simulink model "pam_enlace_simulink"  (R2026a)
settings: Solver=ode23tb  StopTime=T_sim  MaxStep=1e-6  RelTol=1e-4
PostLoadFcn:
  | run(fullfile(fileparts(get_param(bdroot,'FileName')),'pam_simulink_init.m'))
InitFcn:
  | run(fullfile(fileparts(get_param(bdroot,'FileName')),'pam_simulink_init.m'))
values from neighbouring files (symbols this model uses):
  bc = cal.bc    [pam_simulink_init.m]
  den_canal = P.den    [pam_simulink_init.m]
  hc = fliplr(pc) / Ec    [pam_simulink_init.m]
  num_canal = P.num    [pam_simulink_init.m]
  t0 = 3.125e-6    (= 3.125e-06)    [pam_simulink_init.m]
  t_fim = t0 + 7*Tsa    [pam_simulink_init.m]
  t_kstar = t0 + kstar*Tsa    [pam_simulink_init.m]
  tab_bits = zeros(4)    [pam_simulink_init.m]
  thr_u = [cal.thr_u, inf(1, 3 - numel(cal.thr_u))]    [pam_simulink_init.m]
  thr_z = [cal.thr_z, inf(1, 3 - numel(cal.thr_z))]    [pam_simulink_init.m]
  Ts = P.Ts    [pam_simulink_init.m]
  Tsa = P.Tsa    [pam_simulink_init.m]
  Vmax = 3.3    [pam_simulink_init.m]
  Vref = 3.3    [pam_simulink_init.m]
undefined symbols (not defined in the file or in its folder): M, sigma_ruido
settings Model: Creator=fonfon  LastModifiedBy=fonfon

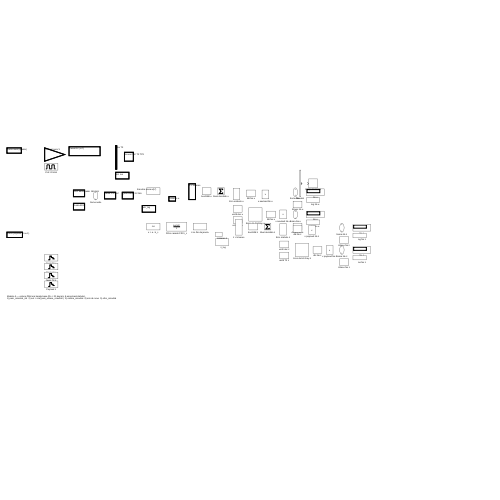
[thumbnail: Simulink's stored preview of the top-level diagram]
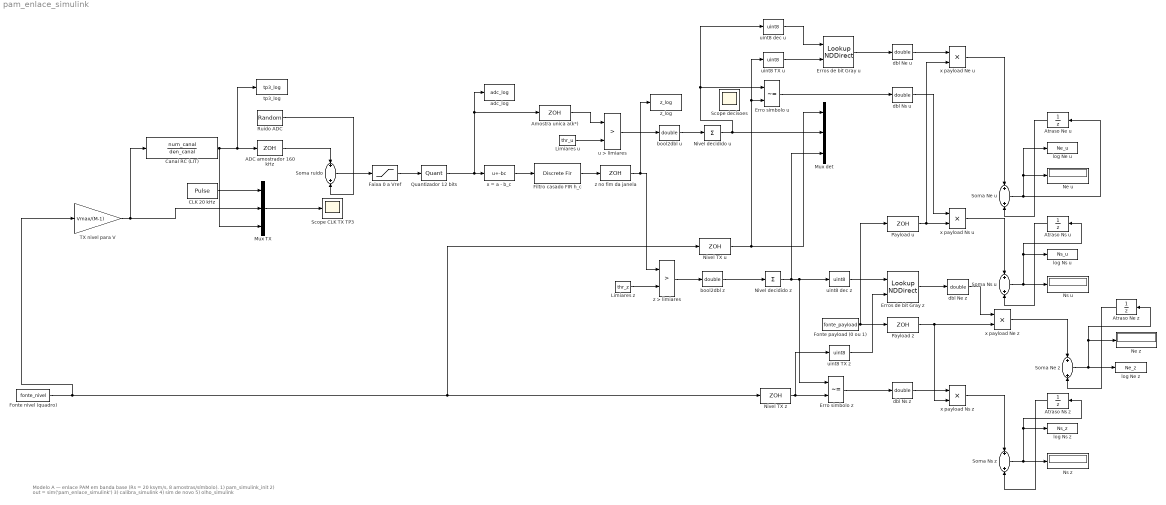
== system pam_enlace_simulink ==
  note: Modelo A — enlace PAM em banda base (Rs = 20 ksym/s, 8 amostras/símbolo).
      | 1) pam_simulink_init  2) out = sim('pam_enlace_simulink')  3) calibra_simulink  4) sim de novo  5) olho_simulink
  ADC amostrador 160 kHz : ZeroOrderHold  SampleTime=[Tsa t0]
  Amostra unica a(k*) : ZeroOrderHold  SampleTime=[Ts t_kstar]
  Atraso Ne u : UnitDelay  SampleTime=-1
  Atraso Ne z : UnitDelay  SampleTime=-1
  Atraso Ns u : UnitDelay  SampleTime=-1
  Atraso Ns z : UnitDelay  SampleTime=-1
  CLK 20 kHz : DiscretePulseGenerator  PulseType=Time based  Amplitude=3.3  Period=Ts  PulseWidth=50
  Canal RC (LIT) : TransferFcn  Numerator=num_canal  Denominator=den_canal
  Erro simbolo u : RelationalOperator  Operator=~=  OutDataTypeStr=boolean  RndMeth=Simplest  InputSameDT=off
  Erro simbolo z : RelationalOperator  Operator=~=  OutDataTypeStr=boolean  RndMeth=Simplest  InputSameDT=off
  Erros de bit Gray u : LookupNDDirect  Table=tab_bits
  Erros de bit Gray z : LookupNDDirect  Table=tab_bits
  Faixa 0 a Vref : Saturate  UpperLimit=Vref  LowerLimit=0
  Filtro casado FIR h_c : DiscreteFir  Coefficients=hc
  Fonte nivel (quadro) : FromWorkspace  VariableName=fonte_nivel  SampleTime=Ts  Interpolate=off  OutputAfterFinalValue=Holding final value
  Fonte payload (0 ou 1) : FromWorkspace  VariableName=fonte_payload  SampleTime=Ts  Interpolate=off  OutputAfterFinalValue=Holding final value
  Limiares u : Constant  Value=thr_u
  Limiares z : Constant  Value=thr_z
  Mux TX : Mux  Inputs=3
  Mux det : Mux  Inputs=3
  Ne u : Display
  Ne z : Display
  Nivel TX u : ZeroOrderHold  SampleTime=[Ts t_kstar]
  Nivel TX z : ZeroOrderHold  SampleTime=[Ts t_fim]
  Nivel decidido u : Sum  Inputs=+
  Nivel decidido z : Sum  Inputs=+
  Ns u : Display
  Ns z : Display
  Payload u : ZeroOrderHold  SampleTime=[Ts t_kstar]
  Payload z : ZeroOrderHold  SampleTime=[Ts t_fim]
  Quantizador 12 bits : Quantizer  QuantizationInterval=q_adc
  Ruido ADC : RandomNumber  Variance=sigma_ruido^2  Seed=1  SampleTime=[Tsa t0]
  Scope CLK TX TP3 : Scope
  Scope decisoes : Scope
  Soma Ne u : Sum
  Soma Ne z : Sum
  Soma Ns u : Sum
  Soma Ns z : Sum
  Soma ruido : Sum
  TX nivel para V : Gain  Gain=Vmax/(M-1)
  adc_log : ToWorkspace  VariableName=adc_log  SampleTime=-1
  bool2dbl u : DataTypeConversion  OutDataTypeStr=double  SaturateOnIntegerOverflow=off  RndMeth=Floor
  bool2dbl z : DataTypeConversion  OutDataTypeStr=double  SaturateOnIntegerOverflow=off  RndMeth=Floor
  dbl Ne u : DataTypeConversion  OutDataTypeStr=double  SaturateOnIntegerOverflow=off  RndMeth=Floor
  dbl Ne z : DataTypeConversion  OutDataTypeStr=double  SaturateOnIntegerOverflow=off  RndMeth=Floor
  dbl Ns u : DataTypeConversion  OutDataTypeStr=double  SaturateOnIntegerOverflow=off  RndMeth=Floor
  dbl Ns z : DataTypeConversion  OutDataTypeStr=double  SaturateOnIntegerOverflow=off  RndMeth=Floor
  log Ne u : ToWorkspace  VariableName=Ne_u  SampleTime=-1
  log Ne z : ToWorkspace  VariableName=Ne_z  SampleTime=-1
  log Ns u : ToWorkspace  VariableName=Ns_u  SampleTime=-1
  log Ns z : ToWorkspace  VariableName=Ns_z  SampleTime=-1
  tp3_log : ToWorkspace  VariableName=tp3_log  SampleTime=0.5e-6
  u > limiares : RelationalOperator  Operator=>  OutDataTypeStr=boolean  RndMeth=Simplest  InputSameDT=off
  uint8 TX u : DataTypeConversion  OutDataTypeStr=uint8  SaturateOnIntegerOverflow=off  RndMeth=Floor
  uint8 TX z : DataTypeConversion  OutDataTypeStr=uint8  SaturateOnIntegerOverflow=off  RndMeth=Floor
  uint8 dec u : DataTypeConversion  OutDataTypeStr=uint8  SaturateOnIntegerOverflow=off  RndMeth=Floor
  uint8 dec z : DataTypeConversion  OutDataTypeStr=uint8  SaturateOnIntegerOverflow=off  RndMeth=Floor
  x = a - b_c : Bias  Bias=-bc  SaturateOnIntegerOverflow=off
  x payload Ne u : Product
  x payload Ne z : Product
  x payload Ns u : Product
  x payload Ns z : Product
  z > limiares : RelationalOperator  Operator=>  OutDataTypeStr=boolean  RndMeth=Simplest  InputSameDT=off
  z no fim da janela : ZeroOrderHold  SampleTime=[Ts t_fim]
  z_log : ToWorkspace  VariableName=z_log  SampleTime=-1
  wires:
  Atraso Ns z/1 -> Soma Ns z/2
  Atraso Ns u/1 -> Soma Ns u/2
  Atraso Ne u/1 -> Soma Ne u/2
  x payload Ns u/1 -> Soma Ns u/1
  dbl Ns u/1 -> x payload Ns u/1
  x payload Ne u/1 -> Soma Ne u/1
  dbl Ne u/1 -> x payload Ne u/1
  Erro simbolo z/1 -> dbl Ns z/1
  uint8 TX z/1 -> Erros de bit Gray z/2
  Soma Ne u/1 -> log Ne u/1, Ne u/1, Atraso Ne u/1
  Limiares u/1 -> u > limiares/2
  Quantizador 12 bits/1 -> adc_log/1, Amostra unica a(k*)/1, x = a - b_c/1
  Soma Ne z/1 -> Ne z/1, Atraso Ne z/1, log Ne z/1
  Soma Ns u/1 -> log Ns u/1, Atraso Ns u/1, Ns u/1
  Faixa 0 a Vref/1 -> Quantizador 12 bits/1
  Mux TX/1 -> Scope CLK TX TP3/1
  x = a - b_c/1 -> Filtro casado FIR h_c/1
  x payload Ns z/1 -> Soma Ns z/1
  Payload z/1 -> x payload Ns z/2, x payload Ne z/2
  ADC amostrador 160 kHz/1 -> Soma ruido/1
  x payload Ne z/1 -> Soma Ne z/1
  Fonte nivel (quadro)/1 -> Nivel TX u/1, Nivel TX z/1, TX nivel para V/1
  Erro simbolo u/1 -> dbl Ns u/1
  Fonte payload (0 ou 1)/1 -> Payload z/1, Payload u/1
  Ruido ADC/1 -> Soma ruido/2
  Canal RC (LIT)/1 -> ADC amostrador 160 kHz/1, tp3_log/1, Mux TX/3
  Filtro casado FIR h_c/1 -> z no fim da janela/1
  Erros de bit Gray z/1 -> dbl Ne z/1
  TX nivel para V/1 -> Canal RC (LIT)/1, Mux TX/2
  Amostra unica a(k*)/1 -> u > limiares/1
  u > limiares/1 -> bool2dbl u/1
  CLK 20 kHz/1 -> Mux TX/1
  z no fim da janela/1 -> z > limiares/1, z_log/1
  Payload u/1 -> x payload Ne u/2, x payload Ns u/2
  Limiares z/1 -> z > limiares/2
  bool2dbl u/1 -> Nivel decidido u/1
  z > limiares/1 -> bool2dbl z/1
  uint8 TX u/1 -> Erros de bit Gray u/2
  Nivel decidido u/1 -> Erro simbolo u/1, uint8 dec u/1, Mux det/2
  Soma Ns z/1 -> log Ns z/1, Atraso Ns z/1, Ns z/1
  Nivel TX u/1 -> Erro simbolo u/2, uint8 TX u/1, Mux det/1
  bool2dbl z/1 -> Nivel decidido z/1
  uint8 dec u/1 -> Erros de bit Gray u/1
  Nivel TX z/1 -> uint8 TX z/1, Erro simbolo z/2
  dbl Ne z/1 -> x payload Ne z/1
  dbl Ns z/1 -> x payload Ns z/1
  Soma ruido/1 -> Faixa 0 a Vref/1
  Nivel decidido z/1 -> Erro simbolo z/1, uint8 dec z/1, Mux det/3
  Erros de bit Gray u/1 -> dbl Ne u/1
  Atraso Ne z/1 -> Soma Ne z/2
  uint8 dec z/1 -> Erros de bit Gray z/1
